simulink model "radio_FM_simulink"  (R2024b)
settings: Solver=FixedStepDiscrete  StartTime=0.0  StopTime=1  FixedStep=sampling_time  RelTol=1e-3  AbsTol=1e-5
values from neighbouring files (symbols this model uses):
  df = beta*W    (= 450)    [parametros.m]
  fc = f_rx    (= 100000)    [parametros.m]
  flo = fc + fi    (= 117000)    [parametros.m]
  sampling_time = 2e-6    (= 2e-06)    [parametros.m]
undefined symbols (not defined in the file or in its folder): dfilt, DiscIntNeverNeededParam
libraries: dspfdesign x7, dsparch4 x2, simulink x1
settings Model: Creator=henao  LastModifiedBy=henao

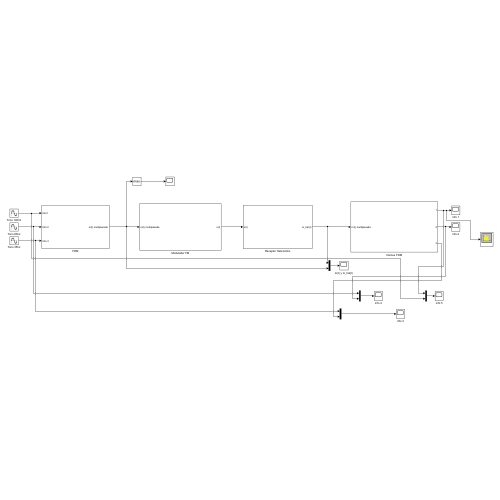
[thumbnail: Simulink's stored preview of the top-level diagram]
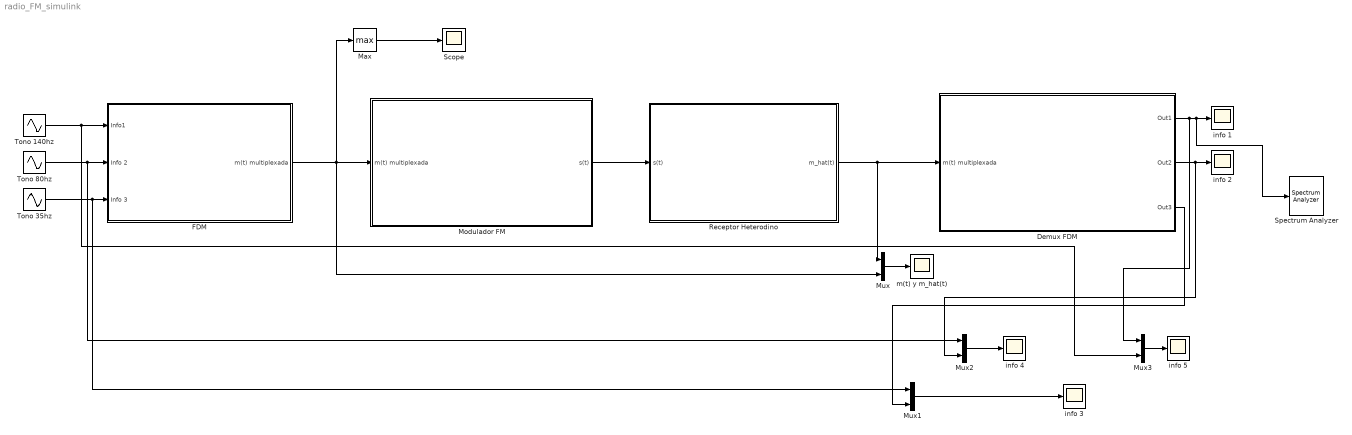
== system radio_FM_simulink ==
  Demux FDM : Subsystem
  FDM : Subsystem
  Max : MinMax  Function=max
  Modulador FM : Subsystem
  Mux{,1..3} (4 alike) : Mux  Inputs=2
  Receptor Heterodino : Subsystem
  Scope : Scope
  Spectrum Analyzer : SpectrumAnalyzer  WindowPosition=[0.000000,36.000000,1440.000000,829.000000,]  Visible=on  ScopeFrameLocation=window  Method=Welch  PlotAsTwoSidedSpectrum=off  FrequencySpan=Start and stop frequencies  StartFrequency=0  StopFrequency=1200  AveragingMethod=Exponential  YLimits=[-90.69910067,30.23298523]
  Tono 140hz : Sin  Frequency=140*2*pi  SampleTime=sampling_time
  Tono 35hz : Sin  Frequency=35*2*pi  SampleTime=sampling_time
  Tono 80hz : Sin  Frequency=80*2*pi  SampleTime=sampling_time
  info {1..5} (5 alike) : Scope
  m(t) y m_hat(t) : Scope
  wires:
  Tono 80hz/1 -> Mux2/1, FDM/2(Info 2)
  Tono 35hz/1 -> Mux1/1, FDM/3(Info 3)
  FDM/1("m(t) multiplexada ") -> Mux/2, Max/1, Modulador FM/1("m(t) multiplexada ")
  Max/1 -> Scope/1
  Modulador FM/1(s(t)) -> Receptor Heterodino/1(s(t))
  Mux/1 -> m(t) y m_hat(t)/1
  Demux FDM/1(Out1) -> Mux3/1, Spectrum Analyzer/1, info 1/1
  Demux FDM/2(Out2) -> Mux2/2, info 2/1
  Demux FDM/3(Out3) -> Mux1/2
  Mux1/1 -> info 3/1
  Mux2/1 -> info 4/1
  Tono 140hz/1 -> Mux3/2, FDM/1(Info1)
  Mux3/1 -> info 5/1
  Receptor Heterodino/1(m_hat(t)) -> Mux/1, Demux FDM/1("m(t) multiplexada ")

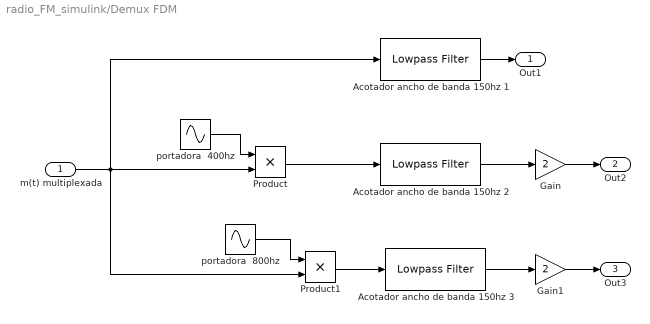
== system radio_FM_simulink/Demux FDM ==
  "m(t) multiplexada " : Inport
  Acotador ancho de banda 150hz 1 : dspfdesign/Lowpass Filter  FilterType=IIR  DesignForMinimumOrder=on  FilterOrder=50  PassbandFrequency=150  StopbandFrequency=170  PassbandRipple=0.1  StopbandAttenuation=40  SampleRateMode=Specify on dialog  SampleRate=sampling_frec  SimulateUsing=Interpreted execution  roundingMode=Floor  coeffsDataTypeStr=fixdt(1,16)
  Acotador ancho de banda 150hz 2 : dspfdesign/Lowpass Filter  FilterType=IIR  DesignForMinimumOrder=on  FilterOrder=50  PassbandFrequency=150  StopbandFrequency=170  PassbandRipple=0.1  StopbandAttenuation=40  SampleRateMode=Specify on dialog  SampleRate=sampling_frec  SimulateUsing=Interpreted execution  roundingMode=Floor  coeffsDataTypeStr=fixdt(1,16)
  Acotador ancho de banda 150hz 3 : dspfdesign/Lowpass Filter  FilterType=IIR  DesignForMinimumOrder=on  FilterOrder=50  PassbandFrequency=150  StopbandFrequency=170  PassbandRipple=0.1  StopbandAttenuation=40  SampleRateMode=Specify on dialog  SampleRate=sampling_frec  SimulateUsing=Interpreted execution  roundingMode=Floor  coeffsDataTypeStr=fixdt(1,16)
  Gain : Gain  Gain=2
  Gain1 : Gain  Gain=2
  Product : Product
  Product1 : Product
  portadora  400hz : Sin  Frequency=400 * 2 * pi  Phase=pi/2 - 400 * 2 * pi*532e-6  SampleTime=sampling_time
  portadora  800hz : Sin  Frequency=800 * 2 * pi  Phase=pi/2- 800 * 2 * pi*532e-6  SampleTime=sampling_time
  Out1 : Outport
  Out2 : Outport  Port=2
  Out3 : Outport  Port=3
  wires:
  portadora  400hz/1 -> Product/1
  Acotador ancho de banda 150hz 1/1 -> Out1/1
  Product/1 -> Acotador ancho de banda 150hz 2/1
  portadora  800hz/1 -> Product1/1
  "m(t) multiplexada "/1 -> Product1/2, Product/2, Acotador ancho de banda 150hz 1/1
  Product1/1 -> Acotador ancho de banda 150hz 3/1
  Acotador ancho de banda 150hz 2/1 -> Gain/1
  Acotador ancho de banda 150hz 3/1 -> Gain1/1
  Gain/1 -> Out2/1
  Gain1/1 -> Out3/1

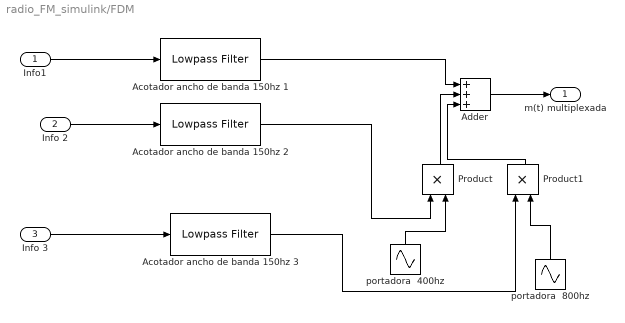
== system radio_FM_simulink/FDM ==
  Info1 : Inport
  Info 2 : Inport  Port=2
  Info 3 : Inport  Port=3
  Acotador ancho de banda 150hz 1 : dspfdesign/Lowpass Filter  FilterType=IIR  DesignForMinimumOrder=on  FilterOrder=50  PassbandFrequency=150  StopbandFrequency=170  PassbandRipple=0.1  StopbandAttenuation=20  SampleRateMode=Specify on dialog  SampleRate=sampling_frec  SimulateUsing=Interpreted execution  roundingMode=Floor  coeffsDataTypeStr=fixdt(1,16)
  Acotador ancho de banda 150hz 2 : dspfdesign/Lowpass Filter  FilterType=IIR  DesignForMinimumOrder=on  FilterOrder=50  PassbandFrequency=150  StopbandFrequency=170  PassbandRipple=0.1  StopbandAttenuation=20  SampleRateMode=Specify on dialog  SampleRate=sampling_frec  SimulateUsing=Interpreted execution  roundingMode=Floor  coeffsDataTypeStr=fixdt(1,16)
  Acotador ancho de banda 150hz 3 : dspfdesign/Lowpass Filter  FilterType=IIR  DesignForMinimumOrder=on  FilterOrder=50  PassbandFrequency=150  StopbandFrequency=170  PassbandRipple=0.1  StopbandAttenuation=20  SampleRateMode=Specify on dialog  SampleRate=sampling_frec  SimulateUsing=Interpreted execution  roundingMode=Floor  coeffsDataTypeStr=fixdt(1,16)
  Adder : Sum  Inputs=+++
  Product : Product
  Product1 : Product
  portadora  400hz : Sin  Frequency=400 * 2 * pi  Phase=pi/2  SampleTime=sampling_time
  portadora  800hz : Sin  Frequency=800 * 2 * pi  Phase=pi/2  SampleTime=sampling_time
  "m(t) multiplexada " : Outport
  wires:
  Acotador ancho de banda 150hz 2/1 -> Product/1
  Product/1 -> Adder/2
  portadora  800hz/1 -> Product1/2
  portadora  400hz/1 -> Product/2
  Acotador ancho de banda 150hz 3/1 -> Product1/1
  Product1/1 -> Adder/3
  Info 2/1 -> Acotador ancho de banda 150hz 2/1
  Info 3/1 -> Acotador ancho de banda 150hz 3/1
  Adder/1 -> "m(t) multiplexada "/1
  Info1/1 -> Acotador ancho de banda 150hz 1/1
  Acotador ancho de banda 150hz 1/1 -> Adder/1

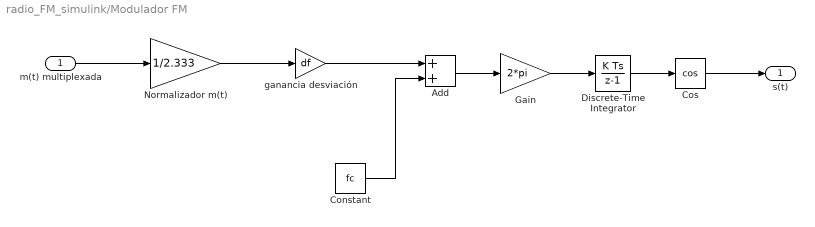
== system radio_FM_simulink/Modulador FM ==
  "m(t) multiplexada " : Inport
  Add : Sum
  Constant : Constant  Value=fc  SampleTime=sampling_time
  Cos : Trigonometry  Operator=cos
  Discrete-Time Integrator : DiscreteIntegrator  SampleTime=sampling_time  ICPrevOutput=DiscIntNeverNeededParam  ICPrevScaledInput=DiscIntNeverNeededParam
  Gain : Gain  Gain=2*pi
  Normalizador m(t) : Gain  Gain=1/2.333
  ganancia desviación : Gain  Gain=df
  s(t) : Outport
  wires:
  Discrete-Time Integrator/1 -> Cos/1
  Normalizador m(t)/1 -> ganancia desviación/1
  Cos/1 -> s(t)/1
  Constant/1 -> Add/2
  Add/1 -> Gain/1
  ganancia desviación/1 -> Add/1
  Gain/1 -> Discrete-Time Integrator/1
  "m(t) multiplexada "/1 -> Normalizador m(t)/1

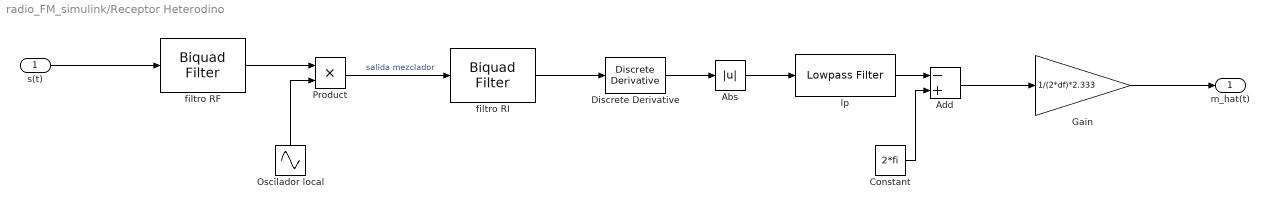
== system radio_FM_simulink/Receptor Heterodino ==
  s(t) : Inport
  Abs : Abs  SaturateOnIntegerOverflow=off
  Add : Sum  Inputs=-+
  Constant : Constant  Value=2*fi
  Discrete Derivative : simulink/Discrete/Discrete Derivative  gainval=1.0  ICPrevScaledInput=0.0  OutMin=[]  OutMax=[]  OutDataType=fixdt(1, 16)  OutScaling=2^-10  DoSatur=off
  Gain : Gain  Gain=1/(2*df)*2.333
  Oscilador local : Sin  Frequency=2*pi*flo  Phase=pi/2  SampleTime=sampling_time
  Product : Product
  filtro RF : dsparch4/Biquad Filter  FilterSource=Dialog parameters  CoeffSource=Specify via dialog  FilterObject=dfilt.df2tsos([1 0.3 0.4],[1 0.1 0.2])  IIRFiltStruct=Direct form II transposed  BiQuadCoeffs=sos_rf  ScaleValues=1  IC=0  ICnum=0  ICden=0  a0Flag=Warning  optimizeScaleValues=on  ScaleValueMode=Specify via input port (g)  roundingMode=Floor  overflowMode=off  scaleValueFracLength=14  denProdOutputFracLength=30  denAccumFracLength=30  secondMemoryFracLength=15
      settings: LibrarySourceBlock=dsphdlsupportfiltering/Biquad Filter
  filtro RI : dsparch4/Biquad Filter  FilterSource=Dialog parameters  CoeffSource=Specify via dialog  FilterObject=dfilt.df2tsos([1 0.3 0.4],[1 0.1 0.2])  IIRFiltStruct=Direct form II transposed  BiQuadCoeffs=sos_fi  ScaleValues=1  IC=0  ICnum=0  ICden=0  a0Flag=Warning  optimizeScaleValues=on  ScaleValueMode=Specify via input port (g)  roundingMode=Floor  overflowMode=off  scaleValueFracLength=14  denProdOutputFracLength=30  denAccumFracLength=30  secondMemoryFracLength=15
      settings: LibrarySourceBlock=dsphdlsupportfiltering/Biquad Filter
  lp : dspfdesign/Lowpass Filter  FilterType=IIR  DesignForMinimumOrder=on  FilterOrder=50  PassbandFrequency=1100  StopbandFrequency=2500  PassbandRipple=0.1  StopbandAttenuation=60  SampleRateMode=Specify on dialog  SampleRate=sampling_frec  SimulateUsing=Interpreted execution  roundingMode=Floor  coeffsDataTypeStr=fixdt(1,16)
  m_hat(t) : Outport
  wires:
  Product/1 -> filtro RI/1  "salida mezclador"
  filtro RF/1 -> Product/1
  filtro RI/1 -> Discrete Derivative/1
  Oscilador local/1 -> Product/2
  s(t)/1 -> filtro RF/1
  Discrete Derivative/1 -> Abs/1
  Abs/1 -> lp/1
  lp/1 -> Add/1
  Constant/1 -> Add/2
  Add/1 -> Gain/1
  Gain/1 -> m_hat(t)/1
